simulink model "PGS_STD_SINV_2STAGE_MODEL_Grid"  (R2024b)
settings: Solver=VariableStepAuto  StartTime=0.0  StopTime=3.0  RelTol=1e-3
PostLoadFcn:
  | gmp_model_file=get_param(bdroot,'FileName'); if isempty(gmp_model_file), error('GMP:SINV:ModelPath', 'The SINV model must be saved before SDPE initialization.'); end; gmp_model_dir=fileparts(gmp_model_file); run(fullfile(gmp_model_dir,'..','..','sdpe_general','sdpe_pgs_sinv_rc_common_settings_matlab_init.m')); run(fullfile(gmp_model_dir,'sdpe_mgr','sdpe_pgs_sinv_rc_simulate_settings_matlab_init.m')); addpath(fullfile(gmp_model_dir,'..','..','..','..','..','tools','gmp_sil','udp_helper_v2','mdl_asio_helper','bin','x64','Debug')); clear gmp_model_file gmp_model_dir;
InitFcn:
  | gmp_model_file=get_param(bdroot,'FileName'); if isempty(gmp_model_file), error('GMP:SINV:ModelPath', 'The SINV model must be saved before SDPE initialization.'); end; gmp_model_dir=fileparts(gmp_model_file); run(fullfile(gmp_model_dir,'..','..','sdpe_general','sdpe_pgs_sinv_rc_common_settings_matlab_init.m')); run(fullfile(gmp_model_dir,'sdpe_mgr','sdpe_pgs_sinv_rc_simulate_settings_matlab_init.m')); addpath(fullfile(gmp_model_dir,'..','..','..','..','..','tools','gmp_sil','udp_helper_v2','mdl_asio_helper','bin','x64','Debug')); clear gmp_model_file gmp_model_dir;
undefined symbols (not defined in the file): CTRL_AC_CURRENT_BIAS, CTRL_AC_CURRENT_SENSITIVITY, CTRL_AC_INDUCTANCE, CTRL_AC_RESISTANCE, CTRL_AC_VOLTAGE_BIAS, CTRL_AC_VOLTAGE_SENSITIVITY, CTRL_ADC_RESOLUTION, CTRL_ADC_VOLTAGE_REF, CTRL_DC_VOLTAGE_BIAS, CTRL_DC_VOLTAGE_SENSITIVITY, CTRL_DCBUS_VOLTAGE, CTRL_GRID_FREQUENCY, CTRL_GRID_VOLTAGE_RMS, CTRL_PWM_CMP_MAX, CTRL_PWM_DEADBAND_CMP, SINV_DC_CAPACITANCE_F, SINV_FILTER_CAP_ESR_OHM, SINV_FILTER_CAPACITANCE_F, SINV_MODEL_DIODE_RON, SINV_MODEL_DIODE_VF, SINV_MODEL_MOSFET_RON, SINV_PWM_FREQUENCY_HZ
libraries: spsSeriesRLCBranchLib x9, spsVoltageMeasurementLib x6, spsSecondOrderFilterLib x5, spsControlledVoltageSourceLib x2, gmp_peripheral_utilities x2, gmp_sil_core_pack x1, spsCurrentMeasurementLib x1, spspowerguiLib x1
settings Model: SimulationMode=accelerator  Creator=javnson  LastModifiedBy=javnson

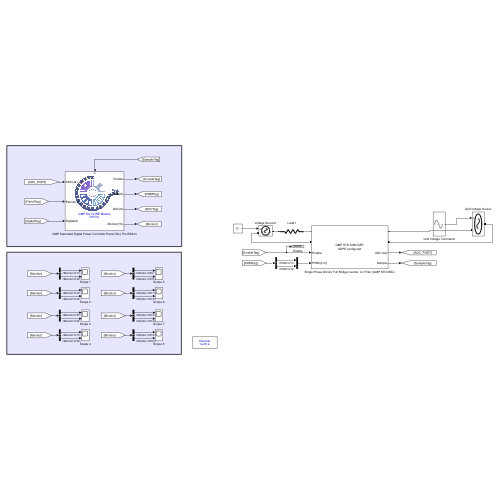
[thumbnail: Simulink's stored preview of the top-level diagram]
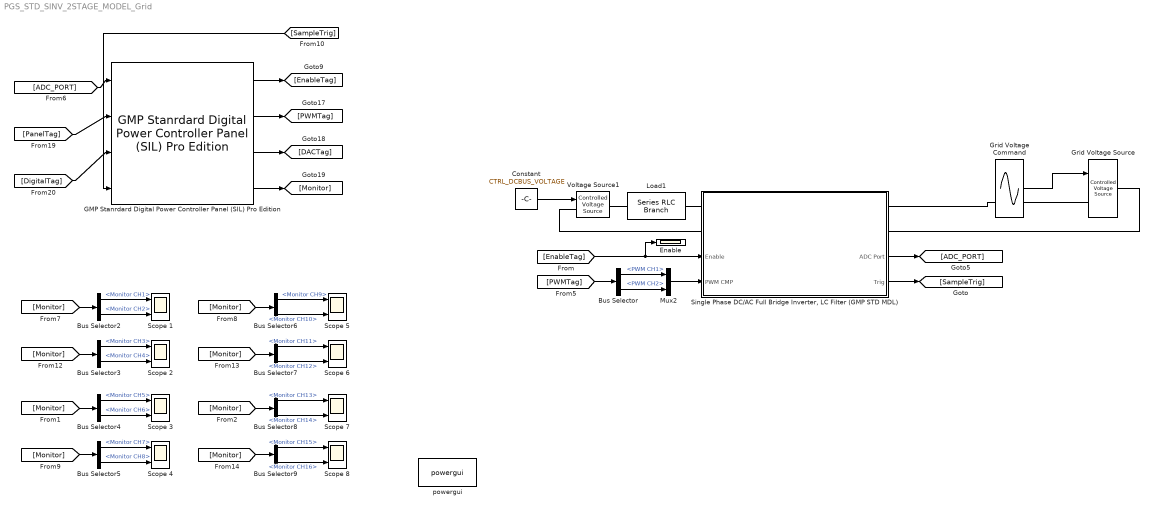
== system PGS_STD_SINV_2STAGE_MODEL_Grid ==
  Bus Selector : BusSelector  OutputSignals=PWM CH1,PWM CH2
  Bus Selector2 : BusSelector  OutputSignals=Monitor CH1,Monitor CH2
  Bus Selector3 : BusSelector  OutputSignals=Monitor CH3,Monitor CH4
  Bus Selector4 : BusSelector  OutputSignals=Monitor CH5,Monitor CH6
  Bus Selector5 : BusSelector  OutputSignals=Monitor CH7,Monitor CH8
  Bus Selector6 : BusSelector  OutputSignals=Monitor CH9,Monitor CH10
  Bus Selector7 : BusSelector  OutputSignals=Monitor CH11,Monitor CH12
  Bus Selector8 : BusSelector  OutputSignals=Monitor CH13,Monitor CH14
  Bus Selector9 : BusSelector  OutputSignals=Monitor CH15,Monitor CH16
  Constant : Constant  Value=CTRL_DCBUS_VOLTAGE
  Enable : Scope
  GMP Stanrdard Digital Power Controller Panel (SIL) Pro Edition : gmp_sil_core_pack/GMP Stanrdard Digital Power Controller Panel (SIL) Pro Edition
      settings: SourceProductName=GMP SIL Core Utilities
  Grid Voltage Command : Sin  Amplitude=sqrt(2) * CTRL_GRID_VOLTAGE_RMS  Frequency=2*pi*CTRL_GRID_FREQUENCY  SampleTime=0
  Grid Voltage Source : spsControlledVoltageSourceLib/Controlled Voltage Source  Initialize=on  Source_Type=AC  Amplitude=0  Phase=0  Frequency=0  Measurements=None
  Load1 : spsSeriesRLCBranchLib/Series RLC Branch  LConnTagsString=__new0  RConnTagsString=__new0  BranchType=R  Resistance=1  Inductance=10e-6  SetiL0=off  InitialCurrent=0  Capacitance=1e-6  Setx0=off  InitialVoltage=0  Measurements=None
  Mux2 : Mux  Inputs=2
  Scope {1..8} (8 alike) : Scope  NumInputPorts=2
  "Single Phase DC/AC Full Bridge Inverter, LC Filter (GMP STD MDL)" : Subsystem  mask(Standard Single Phase DC/AC inverter / rectifier){R_mosfet_on=SINV_MODEL_MOSFET_RON, Lon=0, Rd=SINV_MODEL_DIODE_RON, Vf=SINV_MODEL_DIODE_VF, Rs=1e5, Cs=inf, ACF_L=CTRL_AC_INDUCTANCE, ACF_L_ESR=CTRL_AC_RESISTANCE, ACF_C=SINV_FILTER_CAPACITANCE_F, ACF_C_ESR=SINV_FILTER_CAP_ESR_OHM, ACF_C_EPR=100e3, DC_CAP=SINV_DC_CAPACITANCE_F, DC_CAP_ESR=0.05, DC_CAP_EPR=10e3, fswitch=SINV_PWM_FREQUENCY_HZ, CMP_MAX=CTRL_PWM_CMP_MAX + 1, Deadband_Upper=CTRL_PWM_DEADBAND_CMP, Deadband_Lower=CTRL_PWM_DEADBAND_CMP, phase_shift=0, ADC_Resolution=CTRL_ADC_RESOLUTION, DC_Voltage_Gain=CTRL_DC_VOLTAGE_SENSITIVITY, DC_VOLTAGE_ADC_REFERENCE=CTRL_ADC_VOLTAGE_REF, DC_VOLTAGE_ADC_BIAS=CTRL_DC_VOLTAGE_BIAS, DC_VOLTAGE_ADC_CUT_FREQ=1500, DC_BUS_CURRENT_SENSOR_R=0.02, DC_Current_Gain=20, DC_CURRENT_ADC_REFERENCE=CTRL_ADC_VOLTAGE_REF, DC_CURRENT_ADC_BIAS=CTRL_AC_CURRENT_BIAS, DC_CURRENT_ADC_CUT_FREQ=1500, AC_Voltage_Gain=CTRL_AC_VOLTAGE_SENSITIVITY, AC_VOLTAGE_ADC_REFERENCE=CTRL_ADC_VOLTAGE_REF, AC_VOLTAGE_ADC_BIAS=CTRL_AC_VOLTAGE_BIAS, AC_VOLTAGE_ADC_CUT_FREQ=1500, AC_Current_Gain=CTRL_AC_CURRENT_SENSITIVITY, AC_CURRENT_ADC_REFERENCE=CTRL_ADC_VOLTAGE_REF, AC_CURRENT_ADC_BIAS=CTRL_AC_CURRENT_BIAS, AC_CURRENT_ADC_INIT=0, CAP_CURRENT_SENSOR_R=0.02, CAP_Current_Gain=20, CAP_CURRENT_ADC_REFERENCE=CTRL_ADC_VOLTAGE_REF, CAP_CURRENT_ADC_BIAS=CTRL_AC_CURRENT_BIAS, CAP_CURRENT_ADC_CUT_FREQ=1500, GRID_CURRENT_SENSOR_R=0.02, Grid_Current_Gain=CTRL_AC_CURRENT_SENSITIVITY / 0.02, GRID_CURRENT_ADC_REFERENCE=CTRL_ADC_VOLTAGE_REF, GRID_CURRENT_ADC_BIAS=CTRL_AC_CURRENT_BIAS, GRID_CURRENT_ADC_CUT_FREQ=1500}
      mask prompts: R_mosfet_on "MOSFET on resistance (Ohm)"; Lon "Switch series inductance (H)"; Rd "Body-diode on resistance (Ohm)"; Vf "Body-diode forward voltage (V)"; Rs "Snubber resistance (Ohm)"; Cs "Snubber capacitance (F)"; ACF_L "Series inductance (H)"; ACF_L_ESR "Series resistance (Ohm)"; ACF_C "Shunt capacitance (F)"; ACF_C_ESR "Capacitor ESR (Ohm)"; ACF_C_EPR "Capacitor leakage resistance (Ohm)"; DC_CAP "DC-link capacitance (F)"; DC_CAP_ESR "DC-link capacitor ESR (Ohm)"; DC_CAP_EPR "DC-link leakage resistance (Ohm)"; fswitch "Switching frequency (Hz)"; CMP_MAX "PWM compare full scale"; Deadband_Upper "Upper deadband (counts)"; Deadband_Lower "Lower deadband (counts)"; phase_shift "Carrier phase shift (deg)"; ADC_Resolution "ADC resolution (bits)"; DC_Voltage_Gain "DC voltage sensitivity (V/V)"; DC_VOLTAGE_ADC_REFERENCE "DC voltage ADC reference (V)"; DC_VOLTAGE_ADC_BIAS "DC voltage ADC bias (V)"; DC_VOLTAGE_ADC_CUT_FREQ "DC voltage filter cutoff (Hz)"; DC_BUS_CURRENT_SENSOR_R "DC shunt resistance (Ohm)"; DC_Current_Gain "DC current amplifier gain"; DC_CURRENT_ADC_REFERENCE "DC current ADC reference (V)"; DC_CURRENT_ADC_BIAS "DC current ADC bias (V)"; DC_CURRENT_ADC_CUT_FREQ "DC current filter cutoff (Hz)"; AC_Voltage_Gain "AC voltage sensitivity (V/V)"; AC_VOLTAGE_ADC_REFERENCE "AC voltage ADC reference (V)"; AC_VOLTAGE_ADC_BIAS "AC voltage ADC bias (V)"; AC_VOLTAGE_ADC_CUT_FREQ "AC voltage filter cutoff (Hz)"; AC_Current_Gain "AC current sensitivity (V/A)"; AC_CURRENT_ADC_REFERENCE "AC current ADC reference (V)"; AC_CURRENT_ADC_BIAS "AC current ADC bias (V)"; AC_CURRENT_ADC_INIT "AC current initial value"; CAP_CURRENT_SENSOR_R "Capacitor-current shunt (Ohm)"; CAP_Current_Gain "Capacitor-current amplifier gain"; CAP_CURRENT_ADC_REFERENCE "Capacitor-current ADC reference (V)"; CAP_CURRENT_ADC_BIAS "Capacitor-current ADC bias (V)"; CAP_CURRENT_ADC_CUT_FREQ "Capacitor-current filter cutoff (Hz)"; GRID_CURRENT_SENSOR_R "Grid-current shunt (Ohm)"; Grid_Current_Gain "Grid-current amplifier gain"; GRID_CURRENT_ADC_REFERENCE "Grid-current ADC reference (V)"; GRID_CURRENT_ADC_BIAS "Grid-current ADC bias (V)"; GRID_CURRENT_ADC_CUT_FREQ "Grid-current filter cutoff (Hz)"
      mask help: SDPE-configured single-phase bidirectional converter. ADC bus order: IL, IDC, VDC, IC, VC, IG. PWM order: bridge legs L and N.
      settings: PortSchema="{\"entries\":[{\"content\":{\"sides\":[{\"content\":{\"connectorIds\":[\"LConn1\",\"LConn2\",\"In1\",\"In2\"]},\"type\":\"ConnectorPlacement.EquallySpacedRectSide\",\"uuid\":\"0e3e6e75-5e1a-455b-8a22-c69d0a4261ca\"},{\"content\":{\"connectorIds\":[\"RConn1\",\"RConn2\",\"Out1\",\"Out2\"],\"side\":\"RIGHT\"},\"type\":\"ConnectorPlacement.EquallySpacedRectSide\",\"uuid\":\"20326781-9238-4fea-80fd-ba96906d5d3f\"},{\"content\":{\"side\":\"TOP\"},\"type\":\"ConnectorPlacement.EquallySpacedRectSide\",\"uuid\":\"9e3289d3-0bee-4337-807b-c293a46cda9c\"}]},\"type\":\"ConnectorPlacement.EquallySpacedConnector\",\"uuid\":\"56bb35ad-d602-4874-b9bf-b95a81ef662c\"}],\"packageUris\":[\"http://schema.mathworks.com/mf0/Connector/R2020b\"],\"version\":\"1.0\"}"
      mask DialogControl ParameterGroupVar Prompt: 参数
      mask DialogControl Container4 Prompt: Component Parameters
      mask DialogControl Container7 Prompt: MOSFET
      mask DialogControl Control2 Prompt: Rds(on), unit Ohm
      mask DialogControl Control3 Prompt: Internal diode inducctance, unit H
      mask DialogControl Control4 Prompt: Internal diode resistance Rd, unit Ohm
      mask DialogControl Control5 Prompt: Internal diode forward voltage Vf, unit V
      mask DialogControl Control6 Prompt: Snubber resistance Rs, unit ohm
      mask DialogControl Control7 Prompt: Snubber Capacitance Cs, unit F
      mask DialogControl Container8 Prompt: LC Filter
      mask DialogControl Container20 Prompt: Filter Inductor
      mask DialogControl Control8 Prompt: AC Bus Filter Inductor (H)
      mask DialogControl Control42 Prompt: AC Bus Filter Inductor, ESR (Ohm)
      mask DialogControl Container21 Prompt: Filter Capcitor
      mask DialogControl Control43 Prompt: AC Bus Filter Capacitor (F)
      mask DialogControl Control44 Prompt: AC Bus Filter Capacitor, ESR (Ohm)
      mask DialogControl Control45 Prompt: AC Bus Filter Capacitor, EPR (Ohm)
      mask DialogControl Container22 Prompt: DC Bus Capacitor
      mask DialogControl Control46 Prompt: DC Bus Capacitor (F)
      mask DialogControl Control47 Prompt: DC Bus Capacitor, ESR (Ohm)
      mask DialogControl Control48 Prompt: DC Bus Capacitor, EPR (Ohm)
      mask DialogControl Container5 Prompt: PWM Parameers
      mask DialogControl Control9 Prompt: PWM Frequency (Hz):
      mask DialogControl Control10 Prompt: Full Scale PWM Compare value:
      mask DialogControl Control11 Prompt: (whole period is 2 * CMP_MAX ticks)
      mask DialogControl Control12 Prompt: Deadband Range Set (CMP Value):
      mask DialogControl Control13 Prompt: Single side deadband time: DEADBAND_CMP/2/CMP_MAX/fswitch
      mask DialogControl Control14 Prompt: Initial Phase Shift, unit rad
      mask DialogControl Container6 Prompt: ADC Parameters
      mask DialogControl Container14 Prompt: ADC Device
      mask DialogControl Control15 Prompt: ADC resolution:
      mask DialogControl Container15 Prompt: DC Side Voltage Sensor
      mask DialogControl Control16 Prompt: ADC Voltage Gain (Scale Factor):
      mask DialogControl Control17 Prompt: ADC reference Voltage(V)
      mask DialogControl Control18 Prompt: ADC Bias Voltage(V)
      mask DialogControl Control19 Prompt: Voltage Filter cut frequency (Hz):
      mask DialogControl Control20 Prompt: Generally, this value less than switch frequency / 10, greater than motor normal frequency * 3
      mask DialogControl Container16 Prompt: DC Side Current Sensor
      mask DialogControl Control26 Prompt: DC Bus Current Sensor Resistance
      mask DialogControl Control34 Prompt: ADC Current Gain (Scale Factor):
      mask DialogControl Control27 Prompt: ADC reference Voltage(V), ADC full scale current (when gain = 1)
      mask DialogControl Control28 Prompt: ADC Bias Current(A)
      mask DialogControl Control35 Prompt: Voltage Filter cut frequency (Hz):
      mask DialogControl Control36 Prompt: Generally, this value less than switch frequency / 10, greater than motor normal frequency * 3
      mask DialogControl Container17 Prompt: AC Side Voltage Sensor
      mask DialogControl Control16_copy Prompt: ADC Voltage Gain (Scale Factor):
      mask DialogControl Control17_copy Prompt: ADC reference Voltage(V)
      mask DialogControl Control18_copy Prompt: ADC Bias Voltage(V)
      mask DialogControl Control19_copy Prompt: Voltage Filter cut frequency (Hz):
      mask DialogControl Control20_copy Prompt: Generally, this value less than switch frequency / 10, greater than motor normal frequency * 3
      mask DialogControl Container18 Prompt: AC Side Current Sensor
      mask DialogControl Control26_copy Prompt: ADC Current Gain (Scale Factor):
      mask DialogControl Control27_copy Prompt: ADC reference Current(A), ADC full scale current (when gain = 1)
      mask DialogControl Control28_copy Prompt: ADC Bias Current(A)
      mask DialogControl Control29_copy Prompt: ADC initial Current Output(A)
      mask DialogControl Container19 Prompt: Capcitor Current Sensor
      mask DialogControl Control26_copy_copy Prompt: Filter Capacitor Current Sensor Resistance
      mask DialogControl Control34_copy Prompt: ADC Current Gain (Scale Factor):
      mask DialogControl Control27_copy_copy Prompt: ADC reference Voltage(V), ADC full scale current (when gain = 1)
      mask DialogControl Control28_copy_copy Prompt: ADC Bias Current(V)
      mask DialogControl Control35_copy Prompt: Voltage Filter cut frequency (Hz):
      mask DialogControl Control36_copy Prompt: Generally, this value less than switch frequency / 10, greater than motor normal frequency * 3
      mask DialogControl Container23 Prompt: Grid Current Sensor
      mask DialogControl Control26_copy_copy_copy Prompt: Grid Bus Current Sensor Resistance
      mask DialogControl Control34_copy_copy Prompt: ADC Current Gain (Scale Factor):
      mask DialogControl Control27_copy_copy_copy Prompt: ADC reference Voltage(V), ADC full scale current (when gain = 1)
      mask DialogControl Control28_copy_copy_copy Prompt: ADC Bias Current(V)
      mask DialogControl Control35_copy_copy Prompt: Voltage Filter cut frequency (Hz):
      mask DialogControl Control36_copy_copy Prompt: Generally, this value less than switch frequency / 10, greater than motor normal frequency * 3
      mask DialogControl PWMConfiguration_Group Prompt: PWM Configuration
      mask DialogControl SemiconductorModel_Group Prompt: Semiconductor Model
      mask DialogControl ACFilter_Group Prompt: AC Filter
      mask DialogControl DCLink_Group Prompt: DC Link
      mask DialogControl ADCConfiguration_Group Prompt: ADC Configuration
      mask DialogControl VoltageSensors_Group Prompt: Voltage Sensors
      mask DialogControl CurrentSensors_Group Prompt: Current Sensors
      mask Display:
      | disp('GMP STD SINV/AFE\nSDPE configured');
      | port_label('input',1,'Enable'); port_label('input',2,'PWM [L N]');
      | port_label('output',1,'ADC bus'); port_label('output',2,'Sample');
  Voltage Source1 : spsControlledVoltageSourceLib/Controlled Voltage Source  Initialize=on  Source_Type=AC  Amplitude=0  Phase=0  Frequency=0  Measurements=None
  powergui : spspowerguiLib/powergui  Priority=1  SimulationMode=Discrete  SampleTime=1e-6  frequency=60  Iterations=50  frequencyindice=0  Pbase=100e6  ErrMax=1e-4  UnitsV=kV  UnitsW=MW  buscounter=0  FunctionMessages=off  echomessages=off  EnableUseOfTLC=off  CurrentSourceSwitches=off  DisableSnubberDevices=off  DisableRonSwitches=off  DisableVfSwitches=off  DisplayEquations=off  AutomaticDiscreteSolvers=off  SolverType=Tustin/Backward Euler (TBE)  Interpol=off  ExternalGateDelay=off  methode=off  Ts=100  x0status=blocks  SPID=on  SwTol=0  HookPort=off  NonlinearTolerance=1e-4  nMaxIteration=100  ContinueOnMaxIteration=off  RestoreLinks=warning  ResistiveCurrentMeasurement=off  Frange=[0:2:500]  Ylog=off  Xlog=on  ShowGrid=off  save=off  variable=ZData  structure=0  ZoomFFT=off  StartTime=0.0  cycles=1  DisplayStyle=1  fundamental=60  FreqAxis=off  MaxFrequency=1000  frequencyindicesteady=1  RmsSteady=1  display=off
  wires:
  [PanelTag] -> GMP Stanrdard Digital Power Controller Panel (SIL) Pro Edition/2
  [SampleTrig] -> GMP Stanrdard Digital Power Controller Panel (SIL) Pro Edition/4
  GMP Stanrdard Digital Power Controller Panel (SIL) Pro Edition/2 -> [PWMTag]
  [ADC_PORT] -> GMP Stanrdard Digital Power Controller Panel (SIL) Pro Edition/1
  GMP Stanrdard Digital Power Controller Panel (SIL) Pro Edition/4 -> [Monitor]
  GMP Stanrdard Digital Power Controller Panel (SIL) Pro Edition/1 -> [EnableTag]
  GMP Stanrdard Digital Power Controller Panel (SIL) Pro Edition/3 -> [DACTag]
  [DigitalTag] -> GMP Stanrdard Digital Power Controller Panel (SIL) Pro Edition/3
  [EnableTag] -> "Single Phase DC/AC Full Bridge Inverter, LC Filter (GMP STD MDL)"/1(Enable), Enable/1
  Bus Selector8/2 -> Scope 7/2  "<Monitor CH14>"
  Bus Selector2/2 -> Scope 1/2  "<Monitor CH2>"
  Bus Selector4/2 -> Scope 3/2  "<Monitor CH6>"
  Bus Selector3/1 -> Scope 2/1  "<Monitor CH3>"
  [Monitor] -> Bus Selector4/1
  [Monitor] -> Bus Selector7/1
  Bus Selector2/1 -> Scope 1/1  "<Monitor CH1>"
  Bus Selector5/1 -> Scope 4/1  "<Monitor CH7>"
  [Monitor] -> Bus Selector3/1
  Bus Selector8/1 -> Scope 7/1  "<Monitor CH13>"
  Bus Selector3/2 -> Scope 2/2  "<Monitor CH4>"
  Bus Selector4/1 -> Scope 3/1  "<Monitor CH5>"
  Bus Selector7/1 -> Scope 6/1  "<Monitor CH11>"
  [Monitor] -> Bus Selector5/1
  [Monitor] -> Bus Selector8/1
  [Monitor] -> Bus Selector6/1
  Bus Selector6/1 -> Scope 5/1  "<Monitor CH9>"
  Bus Selector5/2 -> Scope 4/2  "<Monitor CH8>"
  [Monitor] -> Bus Selector2/1
  Bus Selector7/2 -> Scope 6/2  "<Monitor CH12>"
  Bus Selector6/2 -> Scope 5/2  "<Monitor CH10>"
  Bus Selector/1 -> Mux2/1  "<PWM CH1>"
  [PWMTag] -> Bus Selector/1
  Bus Selector9/1 -> Scope 8/1  "<Monitor CH15>"
  [Monitor] -> Bus Selector9/1
  Bus Selector9/2 -> Scope 8/2  "<Monitor CH16>"
  "Single Phase DC/AC Full Bridge Inverter, LC Filter (GMP STD MDL)"/1(ADC Port) -> [ADC_PORT]
  "Single Phase DC/AC Full Bridge Inverter, LC Filter (GMP STD MDL)"/2(Trig) -> [SampleTrig]
  Bus Selector/2 -> Mux2/2  "<PWM CH2>"
  Mux2/1 -> "Single Phase DC/AC Full Bridge Inverter, LC Filter (GMP STD MDL)"/2(PWM CMP)
  Constant/1 -> Voltage Source1/1
  Grid Voltage Command/1 -> Grid Voltage Source/1
  connections:
  Voltage Source1/LConn1 -- "Single Phase DC/AC Full Bridge Inverter, LC Filter (GMP STD MDL)"/LConn2
  Grid Voltage Source/LConn1 -- "Single Phase DC/AC Full Bridge Inverter, LC Filter (GMP STD MDL)"/RConn1
  Grid Voltage Source/RConn1 -- "Single Phase DC/AC Full Bridge Inverter, LC Filter (GMP STD MDL)"/RConn2
  Voltage Source1/RConn1 -- Load1/RConn1
  Load1/LConn1 -- "Single Phase DC/AC Full Bridge Inverter, LC Filter (GMP STD MDL)"/LConn1

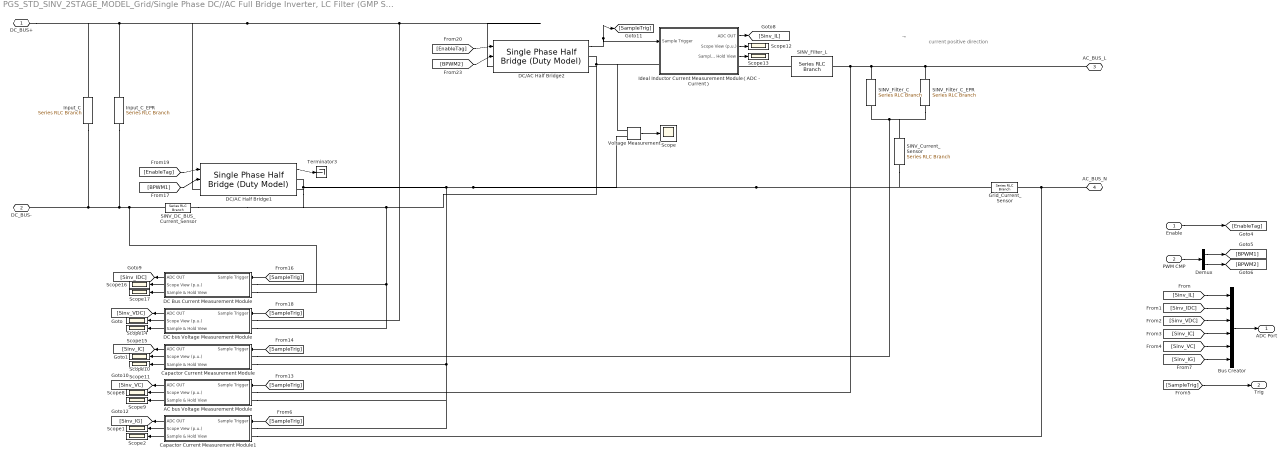
== system PGS_STD_SINV_2STAGE_MODEL_Grid/Single Phase DC//AC Full Bridge Inverter, LC Filter (GMP STD MDL) ==
  note: →
  note: current positive direction
  Enable : Inport
  PWM CMP : Inport  Port=2
  AC bus Voltage Measurement Module : Subsystem  AncestorBlock=peripheral_utilities/Ideal Voltage Measurement with filter Module(ADC - Voltage)  mask{ADC_GAIN=AC_Voltage_Gain, ADC_BIT=ADC_Resolution, ADC_REFERENCE=AC_VOLTAGE_ADC_REFERENCE, ADC_BIAS=AC_VOLTAGE_ADC_BIAS, ADC_INIT=0, cut_frequency=AC_VOLTAGE_ADC_CUT_FREQ}
      mask DialogControl DescGroupVar Prompt: Voltage Sample ADC Model
      mask DialogControl DescTextVar Prompt: This is a ideal Voltage Measurement Module.
      mask DialogControl Control2 Prompt: ADC(p.u.) = (real_voltage * ADC_GAIN + ADC_BIAS)/ADC_REFERENCE
      mask DialogControl Control11 Prompt: GMP CTL Simulink Utilities: virtual peripherals
      mask DialogControl ParameterGroupVar Prompt: Parameters:
      mask DialogControl Control4 Prompt: ADC Voltage Gain (Scale Factor):
      mask DialogControl Control5 Prompt: ADC resolution:
      mask DialogControl Control6 Prompt: ADC reference Voltage(V)
      mask DialogControl Control8 Prompt: ADC Bias Voltage(V)
      mask DialogControl Control7 Prompt: ADC Initial Voltage Output (V):
      mask DialogControl Control9 Prompt: Voltage Filter cut frequency (Hz):
      mask DialogControl Control10 Prompt: Generally, this value less than switch frequency / 10, greater than motor normal frequency * 3
  Bus Creator : BusCreator  Inputs=6
  Capactor Current Measurement Module : Subsystem  AncestorBlock=peripheral_utilities/Ideal Voltage Measurement with filter Module(ADC - Voltage)  mask{ADC_GAIN=CAP_Current_Gain, ADC_BIT=ADC_Resolution, ADC_REFERENCE=CAP_CURRENT_ADC_REFERENCE, ADC_BIAS=CAP_CURRENT_ADC_BIAS, ADC_INIT=0, cut_frequency=CAP_CURRENT_ADC_CUT_FREQ}
      mask DialogControl DescGroupVar Prompt: Voltage Sample ADC Model
      mask DialogControl DescTextVar Prompt: This is a ideal Voltage Measurement Module.
      mask DialogControl Control2 Prompt: ADC(p.u.) = (real_voltage * ADC_GAIN + ADC_BIAS)/ADC_REFERENCE
      mask DialogControl Control11 Prompt: GMP CTL Simulink Utilities: virtual peripherals
      mask DialogControl ParameterGroupVar Prompt: Parameters:
      mask DialogControl Control4 Prompt: ADC Voltage Gain (Scale Factor):
      mask DialogControl Control5 Prompt: ADC resolution:
      mask DialogControl Control6 Prompt: ADC reference Voltage(V)
      mask DialogControl Control8 Prompt: ADC Bias Voltage(V)
      mask DialogControl Control7 Prompt: ADC Initial Voltage Output (V):
      mask DialogControl Control9 Prompt: Voltage Filter cut frequency (Hz):
      mask DialogControl Control10 Prompt: Generally, this value less than switch frequency / 10, greater than motor normal frequency * 3
  Capactor Current Measurement Module1 : Subsystem  AncestorBlock=peripheral_utilities/Ideal Voltage Measurement with filter Module(ADC - Voltage)  mask{ADC_GAIN=Grid_Current_Gain, ADC_BIT=ADC_Resolution, ADC_REFERENCE=GRID_CURRENT_ADC_REFERENCE, ADC_BIAS=GRID_CURRENT_ADC_BIAS, ADC_INIT=0, cut_frequency=GRID_CURRENT_ADC_CUT_FREQ}
      mask DialogControl DescGroupVar Prompt: Voltage Sample ADC Model
      mask DialogControl DescTextVar Prompt: This is a ideal Voltage Measurement Module.
      mask DialogControl Control2 Prompt: ADC(p.u.) = (real_voltage * ADC_GAIN + ADC_BIAS)/ADC_REFERENCE
      mask DialogControl Control11 Prompt: GMP CTL Simulink Utilities: virtual peripherals
      mask DialogControl ParameterGroupVar Prompt: Parameters:
      mask DialogControl Control4 Prompt: ADC Voltage Gain (Scale Factor):
      mask DialogControl Control5 Prompt: ADC resolution:
      mask DialogControl Control6 Prompt: ADC reference Voltage(V)
      mask DialogControl Control8 Prompt: ADC Bias Voltage(V)
      mask DialogControl Control7 Prompt: ADC Initial Voltage Output (V):
      mask DialogControl Control9 Prompt: Voltage Filter cut frequency (Hz):
      mask DialogControl Control10 Prompt: Generally, this value less than switch frequency / 10, greater than motor normal frequency * 3
  DC Bus Current Measurement Module : Subsystem  AncestorBlock=peripheral_utilities/Ideal Voltage Measurement with filter Module(ADC - Voltage)  mask{ADC_GAIN=DC_Current_Gain, ADC_BIT=ADC_Resolution, ADC_REFERENCE=DC_CURRENT_ADC_REFERENCE, ADC_BIAS=DC_CURRENT_ADC_BIAS, ADC_INIT=0, cut_frequency=DC_CURRENT_ADC_CUT_FREQ}
      mask DialogControl DescGroupVar Prompt: Voltage Sample ADC Model
      mask DialogControl DescTextVar Prompt: This is a ideal Voltage Measurement Module.
      mask DialogControl Control2 Prompt: ADC(p.u.) = (real_voltage * ADC_GAIN + ADC_BIAS)/ADC_REFERENCE
      mask DialogControl Control11 Prompt: GMP CTL Simulink Utilities: virtual peripherals
      mask DialogControl ParameterGroupVar Prompt: Parameters:
      mask DialogControl Control4 Prompt: ADC Voltage Gain (Scale Factor):
      mask DialogControl Control5 Prompt: ADC resolution:
      mask DialogControl Control6 Prompt: ADC reference Voltage(V)
      mask DialogControl Control8 Prompt: ADC Bias Voltage(V)
      mask DialogControl Control7 Prompt: ADC Initial Voltage Output (V):
      mask DialogControl Control9 Prompt: Voltage Filter cut frequency (Hz):
      mask DialogControl Control10 Prompt: Generally, this value less than switch frequency / 10, greater than motor normal frequency * 3
  DC bus Voltage Measurement Module : Subsystem  AncestorBlock=peripheral_utilities/Ideal Voltage Measurement with filter Module(ADC - Voltage)  mask{ADC_GAIN=DC_Voltage_Gain, ADC_BIT=ADC_Resolution, ADC_REFERENCE=DC_VOLTAGE_ADC_REFERENCE, ADC_BIAS=DC_VOLTAGE_ADC_BIAS, ADC_INIT=0, cut_frequency=DC_VOLTAGE_ADC_CUT_FREQ}
      mask DialogControl DescGroupVar Prompt: Voltage Sample ADC Model
      mask DialogControl DescTextVar Prompt: This is a ideal Voltage Measurement Module.
      mask DialogControl Control2 Prompt: ADC(p.u.) = (real_voltage * ADC_GAIN + ADC_BIAS)/ADC_REFERENCE
      mask DialogControl Control11 Prompt: GMP CTL Simulink Utilities: virtual peripherals
      mask DialogControl ParameterGroupVar Prompt: Parameters:
      mask DialogControl Control4 Prompt: ADC Voltage Gain (Scale Factor):
      mask DialogControl Control5 Prompt: ADC resolution:
      mask DialogControl Control6 Prompt: ADC reference Voltage(V)
      mask DialogControl Control8 Prompt: ADC Bias Voltage(V)
      mask DialogControl Control7 Prompt: ADC Initial Voltage Output (V):
      mask DialogControl Control9 Prompt: Voltage Filter cut frequency (Hz):
      mask DialogControl Control10 Prompt: Generally, this value less than switch frequency / 10, greater than motor normal frequency * 3
  DC/AC Half Bridge1 : gmp_peripheral_utilities/Single Phase Half Bridge (Duty Model)  fswitch=fswitch  CMP_MAX=CMP_MAX  Deadband_Upper=Deadband_Upper  Deadband_Lower=Deadband_Lower  Deadband_us=NaN  phase_shift=phase_shift  R_mosfet_on=R_mosfet_on  Lon=Lon  Rd=Rd  Vf=Vf  Rs=Rs  Cs=Cs
      settings: SourceProductName=Virtual Peripheral Utilities
  DC/AC Half Bridge2 : gmp_peripheral_utilities/Single Phase Half Bridge (Duty Model)  fswitch=fswitch  CMP_MAX=CMP_MAX  Deadband_Upper=Deadband_Upper  Deadband_Lower=Deadband_Lower  Deadband_us=NaN  phase_shift=phase_shift  R_mosfet_on=R_mosfet_on  Lon=Lon  Rd=Rd  Vf=Vf  Rs=Rs  Cs=Cs
      settings: SourceProductName=Virtual Peripheral Utilities
  Demux : Demux  Outputs=2
  Grid_Current_Sensor : spsSeriesRLCBranchLib/Series RLC Branch  LConnTagsString=__new0  RConnTagsString=__new0  BranchType=R  Resistance=GRID_CURRENT_SENSOR_R  Inductance=1e-3  SetiL0=off  InitialCurrent=0  Capacitance=1e-6  Setx0=off  InitialVoltage=0  Measurements=None
  Ideal Inductor Current Measurement Module（ADC - Current） : Subsystem  AncestorBlock=peripheral_utilities/Ideal Current Measurement Module（ADC - Current）  mask{ADC_GAIN=AC_Current_Gain, ADC_BIT=ADC_Resolution, ADC_REFERENCE=AC_CURRENT_ADC_REFERENCE, ADC_BIAS=AC_CURRENT_ADC_BIAS, ADC_INIT=AC_CURRENT_ADC_INIT}
      mask DialogControl DescGroupVar Prompt: Current Sample ADC Model 1
      mask DialogControl DescTextVar Prompt: This is a ideal Current Measurement Module. This module enable a bias and a gain, and finally output a ADC result.
      mask DialogControl Control8 Prompt: ADC(p.u.) = (real_current * ADC_GAIN + ADC_BIAS)/ADC_REFERENCE
      mask DialogControl Control9 Prompt: GMP CTL Simulink Utilities: virtual peripherals
      mask DialogControl ParameterGroupVar Prompt: 参数
      mask DialogControl Control7 Prompt: ADC Current Gain (Scale Factor):
      mask DialogControl Control2 Prompt: ADC resolution:
      mask DialogControl Control4 Prompt: ADC reference Current(A), ADC full scale current (when gain = 1)
      mask DialogControl Control5 Prompt: ADC Bias Current(A)
      mask DialogControl Control6 Prompt: ADC initial Current Output(A)
  Input_C : spsSeriesRLCBranchLib/Series RLC Branch  LConnTagsString=__new0  RConnTagsString=__new0  BranchType=RC  Resistance=DC_CAP_ESR  Inductance=1e-3  SetiL0=off  InitialCurrent=0  Capacitance=DC_CAP  Setx0=off  InitialVoltage=0  Measurements=None
  Input_C_EPR : spsSeriesRLCBranchLib/Series RLC Branch  LConnTagsString=__new0  RConnTagsString=__new0  BranchType=R  Resistance=DC_CAP_EPR  Inductance=1e-3  SetiL0=off  InitialCurrent=0  Capacitance=1e-6  Setx0=off  InitialVoltage=0  Measurements=None
  SINV_Current_Sensor : spsSeriesRLCBranchLib/Series RLC Branch  LConnTagsString=__new0  RConnTagsString=__new0  BranchType=R  Resistance=CAP_CURRENT_SENSOR_R  Inductance=1e-3  SetiL0=off  InitialCurrent=0  Capacitance=1e-6  Setx0=off  InitialVoltage=0  Measurements=None
  SINV_DC_BUS_Current_Sensor : spsSeriesRLCBranchLib/Series RLC Branch  LConnTagsString=__new0  RConnTagsString=__new0  BranchType=R  Resistance=DC_BUS_CURRENT_SENSOR_R  Inductance=1e-3  SetiL0=off  InitialCurrent=0  Capacitance=1e-6  Setx0=off  InitialVoltage=0  Measurements=None
  SINV_Filter_C : spsSeriesRLCBranchLib/Series RLC Branch  LConnTagsString=__new0  RConnTagsString=__new0  BranchType=RC  Resistance=ACF_C_ESR  Inductance=1e-3  SetiL0=off  InitialCurrent=0  Capacitance=ACF_C  Setx0=off  InitialVoltage=0  Measurements=None
  SINV_Filter_C_EPR : spsSeriesRLCBranchLib/Series RLC Branch  LConnTagsString=__new0  RConnTagsString=__new0  BranchType=R  Resistance=ACF_C_EPR  Inductance=1e-3  SetiL0=off  InitialCurrent=0  Capacitance=1e-6  Setx0=off  InitialVoltage=0  Measurements=None
  SINV_Filter_L : spsSeriesRLCBranchLib/Series RLC Branch  LConnTagsString=__new0  RConnTagsString=__new0  BranchType=RL  Resistance=ACF_L_ESR  Inductance=ACF_L  SetiL0=off  InitialCurrent=0  Capacitance=1e-6  Setx0=off  InitialVoltage=0  Measurements=None
  Scope{,1..2,8..17} (13 alike) : Scope
  Terminator3 : Terminator
  Voltage Measurement : spsVoltageMeasurementLib/Voltage Measurement  PhasorSimulation=off  OutputType=Complex  PSBequivalent=0
  DC_BUS+ : PMIOPort  Side=Left
  DC_BUS- : PMIOPort  Port=2  Side=Left
  AC_BUS_L : PMIOPort  Port=3  Side=Right
  AC_BUS_N : PMIOPort  Port=4  Side=Right
  ADC Port : Outport
  Trig : Outport  Port=2
  wires:
  Voltage Measurement/1 -> Scope/1
  [Sinv_IG] -> Bus Creator/6
  Capactor Current Measurement Module1/3(Sample & Hold View) -> Scope2/1
  Capactor Current Measurement Module1/2(Scope View (p.u.)) -> Scope1/1
  Capactor Current Measurement Module1/1(ADC OUT) -> [Sinv_IG]
  [SampleTrig] -> Capactor Current Measurement Module1/1(Sample Trigger)
  [SampleTrig] -> Trig/1
  Bus Creator/1 -> ADC Port/1
  [Sinv_VC] -> Bus Creator/5
  [Sinv_IC] -> Bus Creator/4
  [Sinv_IL] -> Bus Creator/1
  [Sinv_IDC] -> Bus Creator/2
  [Sinv_VDC] -> Bus Creator/3
  Demux/2 -> [BPWM2]
  Demux/1 -> [BPWM1]
  PWM CMP/1 -> Demux/1
  Enable/1 -> [EnableTag]
  DC Bus Current Measurement Module/1(ADC OUT) -> [Sinv_IDC]
  DC bus Voltage Measurement Module/1(ADC OUT) -> [Sinv_VDC]
  [SampleTrig] -> DC Bus Current Measurement Module/1(Sample Trigger)
  DC bus Voltage Measurement Module/3(Sample & Hold View) -> Scope15/1
  [BPWM1] -> DC/AC Half Bridge1/2
  DC Bus Current Measurement Module/3(Sample & Hold View) -> Scope17/1
  DC bus Voltage Measurement Module/2(Scope View (p.u.)) -> Scope14/1
  Ideal Inductor Current Measurement Module（ADC - Current）/2(Scope View (p.u.)) -> Scope12/1
  Ideal Inductor Current Measurement Module（ADC - Current）/1(ADC OUT) -> [Sinv_IL]
  DC Bus Current Measurement Module/2(Scope View (p.u.)) -> Scope16/1
  Ideal Inductor Current Measurement Module（ADC - Current）/3(Sample & Hold View) -> Scope13/1
  AC bus Voltage Measurement Module/1(ADC OUT) -> [Sinv_VC]
  Capactor Current Measurement Module/1(ADC OUT) -> [Sinv_IC]
  Capactor Current Measurement Module/2(Scope View (p.u.)) -> Scope10/1
  [SampleTrig] -> AC bus Voltage Measurement Module/1(Sample Trigger)
  [SampleTrig] -> Capactor Current Measurement Module/1(Sample Trigger)
  [EnableTag] -> DC/AC Half Bridge1/1
  Capactor Current Measurement Module/3(Sample & Hold View) -> Scope11/1
  [SampleTrig] -> DC bus Voltage Measurement Module/1(Sample Trigger)
  DC/AC Half Bridge1/1 -> Terminator3/1
  [EnableTag] -> DC/AC Half Bridge2/1
  AC bus Voltage Measurement Module/3(Sample & Hold View) -> Scope9/1
  AC bus Voltage Measurement Module/2(Scope View (p.u.)) -> Scope8/1
  [BPWM2] -> DC/AC Half Bridge2/2
  DC/AC Half Bridge2/1 -> [SampleTrig], Ideal Inductor Current Measurement Module（ADC - Current）/1(Sample Trigger)
  connections:
  DC/AC Half Bridge1/RConn1 -- SINV_Current_Sensor/RConn1 -- Grid_Current_Sensor/RConn1 -- Voltage Measurement/LConn2 -- AC bus Voltage Measurement Module/LConn2 -- Capactor Current Measurement Module1/LConn1 -- Capactor Current Measurement Module/LConn2
  DC/AC Half Bridge2/RConn1 -- Voltage Measurement/LConn1 -- Ideal Inductor Current Measurement Module（ADC - Current）/LConn1
  SINV_Filter_L/LConn1 -- Ideal Inductor Current Measurement Module（ADC - Current）/RConn1
  DC bus Voltage Measurement Module/LConn1 -- DC/AC Half Bridge2/LConn1 -- DC/AC Half Bridge1/LConn1 -- DC_BUS+/RConn1 -- Input_C/LConn1 -- Input_C_EPR/LConn1
  AC_BUS_N/RConn1 -- Capactor Current Measurement Module1/LConn2 -- Grid_Current_Sensor/LConn1
  Capactor Current Measurement Module/LConn1 -- SINV_Current_Sensor/LConn1 -- SINV_Filter_C_EPR/RConn1 -- SINV_Filter_C/RConn1
  DC bus Voltage Measurement Module/LConn2 -- DC/AC Half Bridge1/RConn2 -- SINV_DC_BUS_Current_Sensor/LConn1 -- DC/AC Half Bridge2/RConn2 -- DC Bus Current Measurement Module/LConn1
  DC Bus Current Measurement Module/LConn2 -- DC_BUS-/RConn1 -- Input_C/RConn1 -- Input_C_EPR/RConn1 -- SINV_DC_BUS_Current_Sensor/RConn1
  AC_BUS_L/RConn1 -- SINV_Filter_C_EPR/LConn1 -- SINV_Filter_L/RConn1 -- AC bus Voltage Measurement Module/LConn1 -- SINV_Filter_C/LConn1

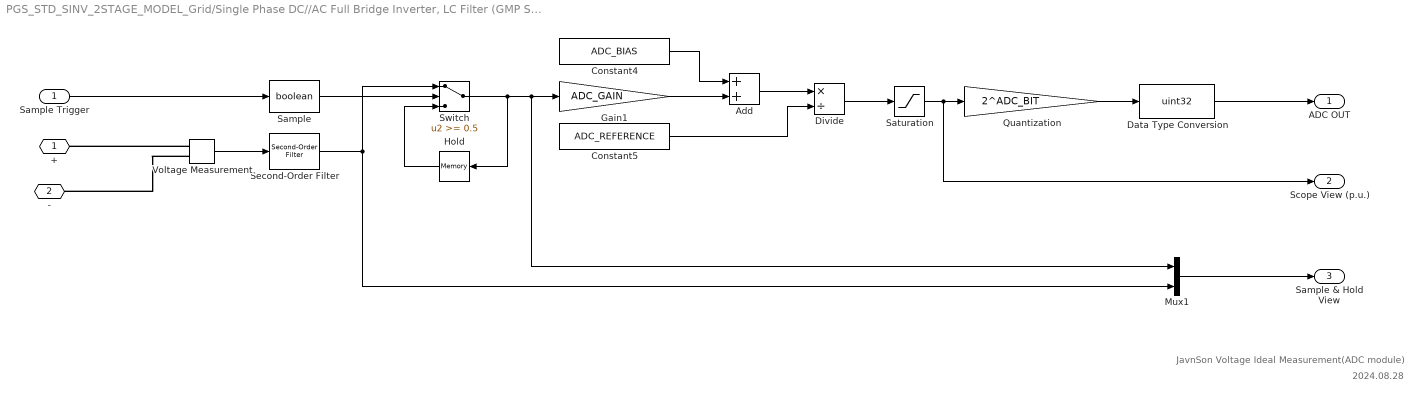
== system PGS_STD_SINV_2STAGE_MODEL_Grid/Single Phase DC//AC Full Bridge Inverter, LC Filter (GMP STD MDL)/AC bus Voltage Measurement Module ==
  note: JavnSon Voltage Ideal Measurement(ADC module)
  note: 2024.08.28
  Sample Trigger : Inport
  Add : Sum
  Constant4 : Constant  Value=ADC_BIAS
  Constant5 : Constant  Value=ADC_REFERENCE
  Data Type Conversion : DataTypeConversion  OutDataTypeStr=uint32  ConvertRealWorld=Stored Integer (SI)  SaturateOnIntegerOverflow=off  RndMeth=Floor
  Divide : Product  Inputs=*/
  Gain1 : Gain  Gain=ADC_GAIN
  Hold : Memory  InitialCondition=ADC_INIT  LinearizeAsDelay=on
  Mux1 : Mux  Inputs=2
  Quantization : Gain  Gain=2^ADC_BIT
  Sample : DataTypeConversion  OutDataTypeStr=boolean  SaturateOnIntegerOverflow=off  RndMeth=Floor
  Saturation : Saturate  UpperLimit=1  LowerLimit=0
  Second-Order Filter : spsSecondOrderFilterLib/Second-Order Filter  FilterType=Lowpass  Fo=cut_frequency  Zeta=0.707  Ts=0  Initialize=off  Vac_Init="[0,  0,  60]"  Vdc_Init=0  PlotResponse=off  FreqRange=[0, 500, 1]
  Switch : Switch  Threshold=0.5
  Voltage Measurement : spsVoltageMeasurementLib/Voltage Measurement  PhasorSimulation=off  OutputType=Complex  PSBequivalent=0
  + : PMIOPort  Side=Left
  - : PMIOPort  Port=2  Side=Left
  ADC OUT : Outport
  Scope View (p.u.) : Outport  Port=2
  Sample & Hold View : Outport  Port=3
  wires:
  Second-Order Filter/1 -> Mux1/2, Switch/1
  Hold/1 -> Switch/3
  Switch/1 -> Hold/1, Mux1/1, Gain1/1
  Divide/1 -> Saturation/1
  Voltage Measurement/1 -> Second-Order Filter/1
  Saturation/1 -> Scope View (p.u.)/1, Quantization/1
  Constant4/1 -> Add/1
  Gain1/1 -> Add/2
  Sample Trigger/1 -> Sample/1
  Data Type Conversion/1 -> ADC OUT/1
  Mux1/1 -> Sample & Hold View/1
  Quantization/1 -> Data Type Conversion/1
  Constant5/1 -> Divide/2
  Add/1 -> Divide/1
  Sample/1 -> Switch/2
  connections:
  Voltage Measurement/LConn1 -- +/RConn1
  Voltage Measurement/LConn2 -- -/RConn1

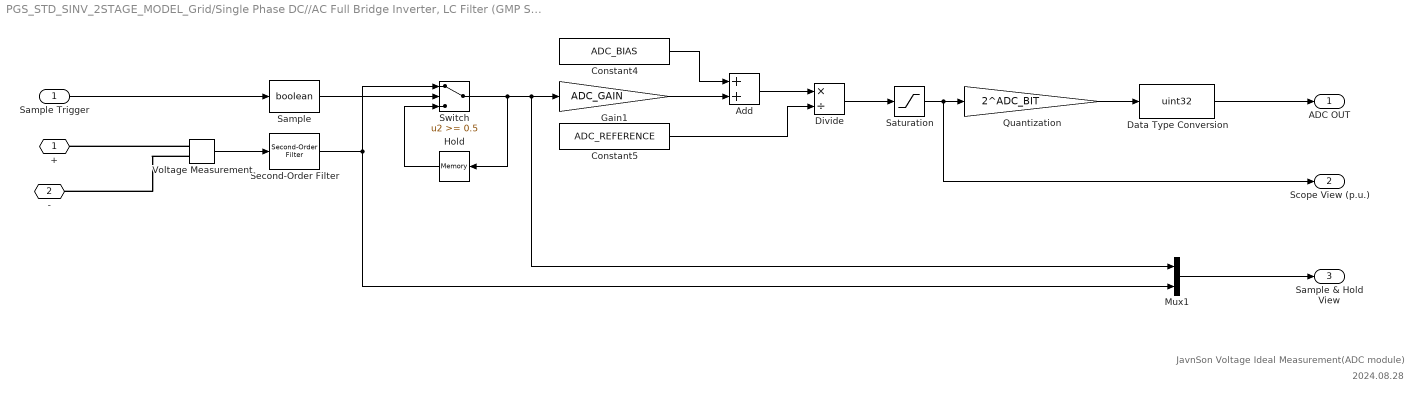
== system PGS_STD_SINV_2STAGE_MODEL_Grid/Single Phase DC//AC Full Bridge Inverter, LC Filter (GMP STD MDL)/Capactor Current Measurement Module ==
  note: 2024.08.28
  note: JavnSon Voltage Ideal Measurement(ADC module)
  Sample Trigger : Inport
  Add : Sum
  Constant4 : Constant  Value=ADC_BIAS
  Constant5 : Constant  Value=ADC_REFERENCE
  Data Type Conversion : DataTypeConversion  OutDataTypeStr=uint32  ConvertRealWorld=Stored Integer (SI)  SaturateOnIntegerOverflow=off  RndMeth=Floor
  Divide : Product  Inputs=*/
  Gain1 : Gain  Gain=ADC_GAIN
  Hold : Memory  InitialCondition=ADC_INIT  LinearizeAsDelay=on
  Mux1 : Mux  Inputs=2
  Quantization : Gain  Gain=2^ADC_BIT
  Sample : DataTypeConversion  OutDataTypeStr=boolean  SaturateOnIntegerOverflow=off  RndMeth=Floor
  Saturation : Saturate  UpperLimit=1  LowerLimit=0
  Second-Order Filter : spsSecondOrderFilterLib/Second-Order Filter  FilterType=Lowpass  Fo=cut_frequency  Zeta=0.707  Ts=0  Initialize=off  Vac_Init="[0,  0,  60]"  Vdc_Init=0  PlotResponse=off  FreqRange=[0, 500, 1]
  Switch : Switch  Threshold=0.5
  Voltage Measurement : spsVoltageMeasurementLib/Voltage Measurement  PhasorSimulation=off  OutputType=Complex  PSBequivalent=0
  + : PMIOPort  Side=Left
  - : PMIOPort  Port=2  Side=Left
  ADC OUT : Outport
  Scope View (p.u.) : Outport  Port=2
  Sample & Hold View : Outport  Port=3
  wires:
  Sample/1 -> Switch/2
  Add/1 -> Divide/1
  Constant5/1 -> Divide/2
  Quantization/1 -> Data Type Conversion/1
  Mux1/1 -> Sample & Hold View/1
  Data Type Conversion/1 -> ADC OUT/1
  Sample Trigger/1 -> Sample/1
  Gain1/1 -> Add/2
  Constant4/1 -> Add/1
  Saturation/1 -> Quantization/1, Scope View (p.u.)/1
  Voltage Measurement/1 -> Second-Order Filter/1
  Divide/1 -> Saturation/1
  Switch/1 -> Gain1/1, Mux1/1, Hold/1
  Hold/1 -> Switch/3
  Second-Order Filter/1 -> Switch/1, Mux1/2
  connections:
  Voltage Measurement/LConn2 -- -/RConn1
  Voltage Measurement/LConn1 -- +/RConn1

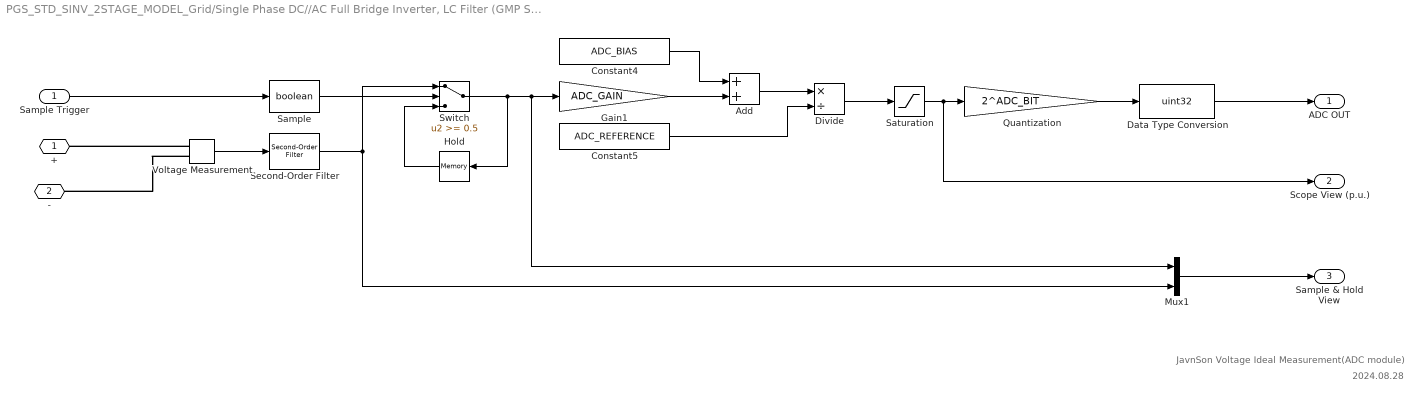
== system PGS_STD_SINV_2STAGE_MODEL_Grid/Single Phase DC//AC Full Bridge Inverter, LC Filter (GMP STD MDL)/Capactor Current Measurement Module1 ==
  note: JavnSon Voltage Ideal Measurement(ADC module)
  note: 2024.08.28
  Sample Trigger : Inport
  Add : Sum
  Constant4 : Constant  Value=ADC_BIAS
  Constant5 : Constant  Value=ADC_REFERENCE
  Data Type Conversion : DataTypeConversion  OutDataTypeStr=uint32  ConvertRealWorld=Stored Integer (SI)  SaturateOnIntegerOverflow=off  RndMeth=Floor
  Divide : Product  Inputs=*/
  Gain1 : Gain  Gain=ADC_GAIN
  Hold : Memory  InitialCondition=ADC_INIT  LinearizeAsDelay=on
  Mux1 : Mux  Inputs=2
  Quantization : Gain  Gain=2^ADC_BIT
  Sample : DataTypeConversion  OutDataTypeStr=boolean  SaturateOnIntegerOverflow=off  RndMeth=Floor
  Saturation : Saturate  UpperLimit=1  LowerLimit=0
  Second-Order Filter : spsSecondOrderFilterLib/Second-Order Filter  FilterType=Lowpass  Fo=cut_frequency  Zeta=0.707  Ts=0  Initialize=off  Vac_Init="[0,  0,  60]"  Vdc_Init=0  PlotResponse=off  FreqRange=[0, 500, 1]
  Switch : Switch  Threshold=0.5
  Voltage Measurement : spsVoltageMeasurementLib/Voltage Measurement  PhasorSimulation=off  OutputType=Complex  PSBequivalent=0
  + : PMIOPort  Side=Left
  - : PMIOPort  Port=2  Side=Left
  ADC OUT : Outport
  Scope View (p.u.) : Outport  Port=2
  Sample & Hold View : Outport  Port=3
  wires:
  Second-Order Filter/1 -> Mux1/2, Switch/1
  Hold/1 -> Switch/3
  Switch/1 -> Hold/1, Mux1/1, Gain1/1
  Divide/1 -> Saturation/1
  Voltage Measurement/1 -> Second-Order Filter/1
  Saturation/1 -> Scope View (p.u.)/1, Quantization/1
  Constant4/1 -> Add/1
  Gain1/1 -> Add/2
  Sample Trigger/1 -> Sample/1
  Data Type Conversion/1 -> ADC OUT/1
  Mux1/1 -> Sample & Hold View/1
  Quantization/1 -> Data Type Conversion/1
  Constant5/1 -> Divide/2
  Add/1 -> Divide/1
  Sample/1 -> Switch/2
  connections:
  Voltage Measurement/LConn1 -- +/RConn1
  Voltage Measurement/LConn2 -- -/RConn1

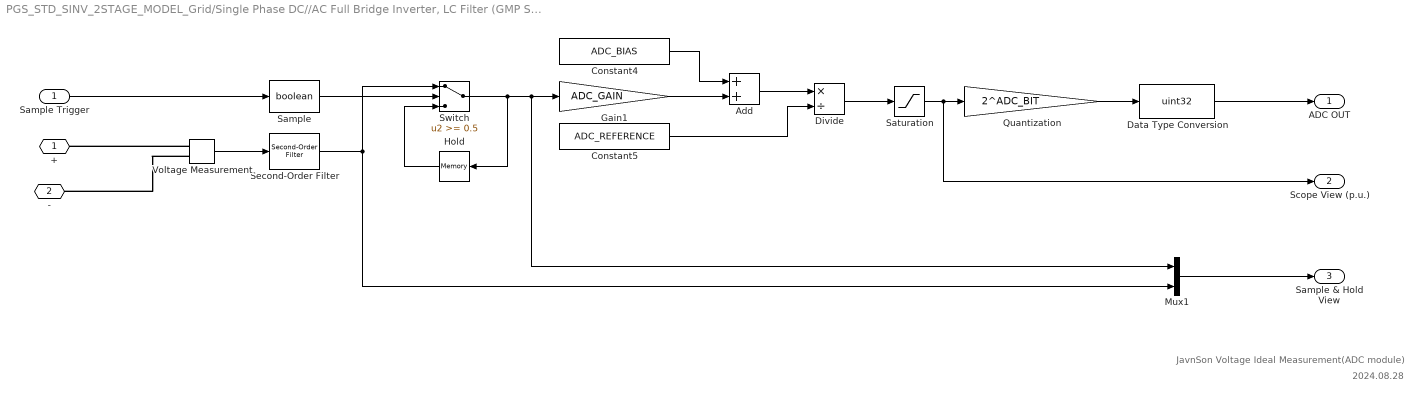
== system PGS_STD_SINV_2STAGE_MODEL_Grid/Single Phase DC//AC Full Bridge Inverter, LC Filter (GMP STD MDL)/DC Bus Current Measurement Module ==
  note: 2024.08.28
  note: JavnSon Voltage Ideal Measurement(ADC module)
  Sample Trigger : Inport
  Add : Sum
  Constant4 : Constant  Value=ADC_BIAS
  Constant5 : Constant  Value=ADC_REFERENCE
  Data Type Conversion : DataTypeConversion  OutDataTypeStr=uint32  ConvertRealWorld=Stored Integer (SI)  SaturateOnIntegerOverflow=off  RndMeth=Floor
  Divide : Product  Inputs=*/
  Gain1 : Gain  Gain=ADC_GAIN
  Hold : Memory  InitialCondition=ADC_INIT  LinearizeAsDelay=on
  Mux1 : Mux  Inputs=2
  Quantization : Gain  Gain=2^ADC_BIT
  Sample : DataTypeConversion  OutDataTypeStr=boolean  SaturateOnIntegerOverflow=off  RndMeth=Floor
  Saturation : Saturate  UpperLimit=1  LowerLimit=0
  Second-Order Filter : spsSecondOrderFilterLib/Second-Order Filter  FilterType=Lowpass  Fo=cut_frequency  Zeta=0.707  Ts=0  Initialize=off  Vac_Init="[0,  0,  60]"  Vdc_Init=0  PlotResponse=off  FreqRange=[0, 500, 1]
  Switch : Switch  Threshold=0.5
  Voltage Measurement : spsVoltageMeasurementLib/Voltage Measurement  PhasorSimulation=off  OutputType=Complex  PSBequivalent=0
  + : PMIOPort  Side=Left
  - : PMIOPort  Port=2  Side=Left
  ADC OUT : Outport
  Scope View (p.u.) : Outport  Port=2
  Sample & Hold View : Outport  Port=3
  wires:
  Sample/1 -> Switch/2
  Add/1 -> Divide/1
  Constant5/1 -> Divide/2
  Quantization/1 -> Data Type Conversion/1
  Mux1/1 -> Sample & Hold View/1
  Data Type Conversion/1 -> ADC OUT/1
  Sample Trigger/1 -> Sample/1
  Gain1/1 -> Add/2
  Constant4/1 -> Add/1
  Saturation/1 -> Quantization/1, Scope View (p.u.)/1
  Voltage Measurement/1 -> Second-Order Filter/1
  Divide/1 -> Saturation/1
  Switch/1 -> Gain1/1, Mux1/1, Hold/1
  Hold/1 -> Switch/3
  Second-Order Filter/1 -> Switch/1, Mux1/2
  connections:
  Voltage Measurement/LConn2 -- -/RConn1
  Voltage Measurement/LConn1 -- +/RConn1

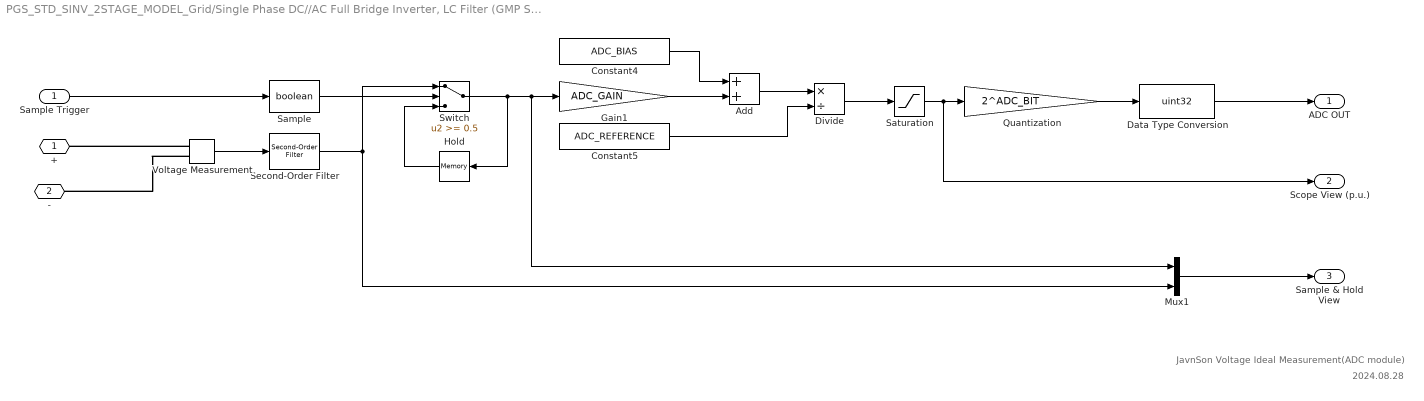
== system PGS_STD_SINV_2STAGE_MODEL_Grid/Single Phase DC//AC Full Bridge Inverter, LC Filter (GMP STD MDL)/DC bus Voltage Measurement Module ==
  note: JavnSon Voltage Ideal Measurement(ADC module)
  note: 2024.08.28
  Sample Trigger : Inport
  Add : Sum
  Constant4 : Constant  Value=ADC_BIAS
  Constant5 : Constant  Value=ADC_REFERENCE
  Data Type Conversion : DataTypeConversion  OutDataTypeStr=uint32  ConvertRealWorld=Stored Integer (SI)  SaturateOnIntegerOverflow=off  RndMeth=Floor
  Divide : Product  Inputs=*/
  Gain1 : Gain  Gain=ADC_GAIN
  Hold : Memory  InitialCondition=ADC_INIT  LinearizeAsDelay=on
  Mux1 : Mux  Inputs=2
  Quantization : Gain  Gain=2^ADC_BIT
  Sample : DataTypeConversion  OutDataTypeStr=boolean  SaturateOnIntegerOverflow=off  RndMeth=Floor
  Saturation : Saturate  UpperLimit=1  LowerLimit=0
  Second-Order Filter : spsSecondOrderFilterLib/Second-Order Filter  FilterType=Lowpass  Fo=cut_frequency  Zeta=0.707  Ts=0  Initialize=off  Vac_Init="[0,  0,  60]"  Vdc_Init=0  PlotResponse=off  FreqRange=[0, 500, 1]
  Switch : Switch  Threshold=0.5
  Voltage Measurement : spsVoltageMeasurementLib/Voltage Measurement  PhasorSimulation=off  OutputType=Complex  PSBequivalent=0
  + : PMIOPort  Side=Left
  - : PMIOPort  Port=2  Side=Left
  ADC OUT : Outport
  Scope View (p.u.) : Outport  Port=2
  Sample & Hold View : Outport  Port=3
  wires:
  Second-Order Filter/1 -> Mux1/2, Switch/1
  Hold/1 -> Switch/3
  Switch/1 -> Hold/1, Mux1/1, Gain1/1
  Divide/1 -> Saturation/1
  Voltage Measurement/1 -> Second-Order Filter/1
  Saturation/1 -> Scope View (p.u.)/1, Quantization/1
  Constant4/1 -> Add/1
  Gain1/1 -> Add/2
  Sample Trigger/1 -> Sample/1
  Data Type Conversion/1 -> ADC OUT/1
  Mux1/1 -> Sample & Hold View/1
  Quantization/1 -> Data Type Conversion/1
  Constant5/1 -> Divide/2
  Add/1 -> Divide/1
  Sample/1 -> Switch/2
  connections:
  Voltage Measurement/LConn1 -- +/RConn1
  Voltage Measurement/LConn2 -- -/RConn1

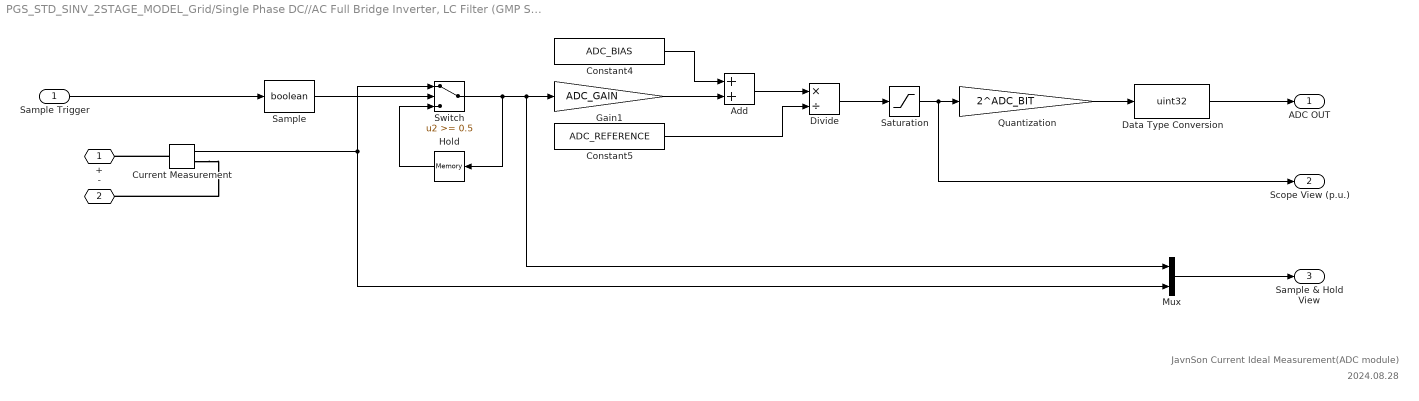
== system PGS_STD_SINV_2STAGE_MODEL_Grid/Single Phase DC//AC Full Bridge Inverter, LC Filter (GMP STD MDL)/Ideal Inductor Current Measurement Module（ADC - Current） ==
  note: JavnSon Current Ideal Measurement(ADC module)
  note: 2024.08.28
  Sample Trigger : Inport
  Add : Sum
  Constant4 : Constant  Value=ADC_BIAS
  Constant5 : Constant  Value=ADC_REFERENCE
  Current Measurement : spsCurrentMeasurementLib/Current Measurement  PhasorSimulation=off  OutputType=Complex  PSBequivalent=0
  Data Type Conversion : DataTypeConversion  OutDataTypeStr=uint32  ConvertRealWorld=Stored Integer (SI)  SaturateOnIntegerOverflow=off  RndMeth=Floor
  Divide : Product  Inputs=*/
  Gain1 : Gain  Gain=ADC_GAIN
  Hold : Memory  InitialCondition=ADC_INIT  LinearizeAsDelay=on
  Mux : Mux  Inputs=2
  Quantization : Gain  Gain=2^ADC_BIT
  Sample : DataTypeConversion  OutDataTypeStr=boolean  SaturateOnIntegerOverflow=off  RndMeth=Floor
  Saturation : Saturate  UpperLimit=1  LowerLimit=0
  Switch : Switch  Threshold=0.5
  + : PMIOPort  Side=Left
  - : PMIOPort  Port=2  Side=Right
  ADC OUT : Outport
  Scope View (p.u.) : Outport  Port=2
  Sample & Hold View : Outport  Port=3
  wires:
  Constant5/1 -> Divide/2
  Quantization/1 -> Data Type Conversion/1
  Sample/1 -> Switch/2
  Add/1 -> Divide/1
  Sample Trigger/1 -> Sample/1
  Data Type Conversion/1 -> ADC OUT/1
  Hold/1 -> Switch/3
  Current Measurement/1 -> Mux/2, Switch/1
  Constant4/1 -> Add/1
  Switch/1 -> Hold/1, Mux/1, Gain1/1
  Gain1/1 -> Add/2
  Saturation/1 -> Scope View (p.u.)/1, Quantization/1
  Divide/1 -> Saturation/1
  Mux/1 -> Sample & Hold View/1
  connections:
  Current Measurement/LConn1 -- +/RConn1
  Current Measurement/RConn1 -- -/RConn1
